simulink model "afe_uvw_ctrl"  (R2026b)
settings: Solver=VariableStepAuto
undefined symbols (not defined in the file or in its folder): param
(part 1 of 2)
settings Model: Creator=pwr-control  LastModifiedBy=d.bagnara

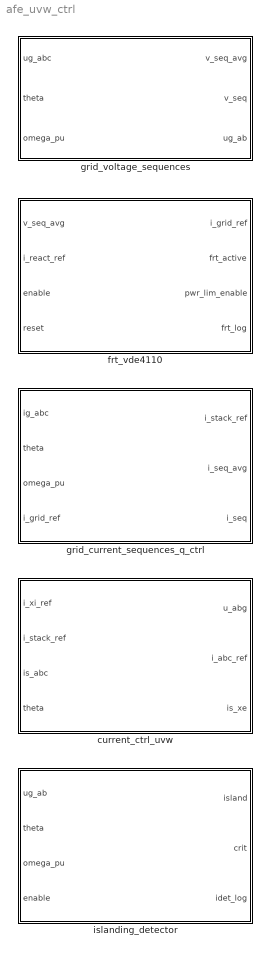
== system afe_uvw_ctrl ==
  current_ctrl_uvw : Subsystem  mask(Per-phase resonant current control (MATLAB Function)){p=param.afe.uvw}
      mask prompts: p "Parameter struct p (see afe_uvw_ctrl_param_example.m)"
      mask help: Current control of the stack (converter) current, one resonant PI per phase: the references of the sequence frames (xi from the DC-link control, [pos_eta; neg_xi; neg_eta] from grid_current_sequences_q_ctrl) become three phase current references; per phase d = kp*e + ki*s/(s^2 + 2*delta*w*s + w^2)*e (forward-backward Euler with p.ts: the new x1 in the update of x2, poles inside the unit circle for delta greater than 0; w = p.ictrl.omega_res, delta = p.ictrl.delta_res); the three outputs are divided by the length of the previous alpha/beta vector (limited to [p.ictrl.mag_lim, p.ictrl.mag_scale_max]) and transformed to alpha/beta, one step late as the model when p.ictrl.out_delay = 1; a PI on the zero-sequence current gives u_gamma. Inputs: i_xi_ref [pu], i_stack_ref [3x1] pu, is_abc [3x1] pu, theta [rad]. Outputs: u_abg [3x1] = [u_alpha; u_beta; u_gamma] pu for the modulator, i_abc_ref [3x1] pu, is_xe [2x1] = [xi; eta] stack current in the positive frame (log). MATLAB Function version of the subsystem current_ctrl of the model afe_uvw_three_phase. Source src/current_ctrl_uvw.m of library/masked_models/afe_uvw_ctrl (update_afe_uvw_ctrl.m loads it into the block). The block inherits its sample time: run it at p.ts (triggered or discrete subsystem clocked at p.ts, as the control of the model, or a fixed-step discrete model). Parameter p: one struct for the five blocks, see afe_uvw_ctrl_param_example.m. User guide: Help of the block (README.md of the folder).
      mask Help: web('https://github.com/pwr-control/library/blob/dev/library/masked_models/afe_uvw_ctrl/README.md', '-browser')
      mask Display:
      | disp(sprintf('per-phase resonant\ncurrent control'))
      | port_label('input', 1, 'i_xi_ref')
      | port_label('input', 2, 'i_stack_ref')
      | port_label('input', 3, 'is_abc')
      | port_label('input', 4, 'theta')
      | port_label('output', 1, 'u_abg')
      | port_label('output', 2, 'i_abc_ref')
      | port_label('output', 3, 'is_xe')
  frt_vde4110 : Subsystem  mask(Fault ride-through VDE-AR-N 4110 (MATLAB Function)){p=param.afe.uvw}
      mask prompts: p "Parameter struct p (see afe_uvw_ctrl_param_example.m)"
      mask help: Fault detection and reactive current references for the fault ride-through. A fault is detected when the positive sequence leaves [p.frt.v_pos_low, p.frt.v_pos_high] or the negative sequence exceeds p.frt.v_neg_max while the voltage changes faster than p.frt.v_pos_dot_max (double-integrator observers); state machine IDLE / ACTIVE / EXCEEDED (fault longer than p.frt.t_hold_max, left with reset). During the fault: pwr_lim_enable when the voltage is below p.frt.pwrlim_v_pos, and i_grid_ref = [pos_eta; neg_xi; neg_eta] = normal reactive references + p.frt.k_frt_ref times the change of the voltage sequences against their pre-fault averages (p.frt.t_avg_prefault, frozen during the fault), limited and low-pass filtered (p.frt.f_lpf_ref). Inputs: v_seq_avg [4x1] from grid_voltage_sequences, i_react_ref [2x1] = [pos; neg] reactive grid current references in normal operation [pu], enable (> 0.5 detector on), reset (> 0.5 leaves EXCEEDED). Outputs: i_grid_ref [3x1] pu -> grid_current_sequences_q_ctrl, frt_active (0/1), pwr_lim_enable (0/1, for the DC-link control), frt_log [10x1] = [state; exceeded; red_dyn; v_pos_dot; v_neg_dot; v_prefault (4); |v_neg|]. MATLAB Function version of the subsystem FRT-VDE4110 of the model afe_uvw_three_phase. Source src/frt_vde4110.m of library/masked_models/afe_uvw_ctrl (update_afe_uvw_ctrl.m loads it into the block). The block inherits its sample time: run it at p.ts (triggered or discrete subsystem clocked at p.ts, as the control of the model, or a fixed-step discrete model). Parameter p: one struct for the five blocks, see afe_uvw_ctrl_param_example.m. User guide: Help of the block (README.md of the folder).
      mask Help: web('https://github.com/pwr-control/library/blob/dev/library/masked_models/afe_uvw_ctrl/README.md', '-browser')
      mask Display:
      | disp(sprintf('fault ride-through\nVDE-AR-N 4110'))
      | port_label('input', 1, 'v_seq_avg')
      | port_label('input', 2, 'i_react_ref')
      | port_label('input', 3, 'enable')
      | port_label('input', 4, 'reset')
      | port_label('output', 1, 'i_grid_ref')
      | port_label('output', 2, 'frt_active')
      | port_label('output', 3, 'pwr_lim_enable')
      | port_label('output', 4, 'frt_log')
  grid_current_sequences_q_ctrl : Subsystem  mask(Grid current sequences and reactive current control (MATLAB Function)){p=param.afe.uvw}
      mask prompts: p "Parameter struct p (see afe_uvw_ctrl_param_example.m)"
      mask help: Sequence components of the grid current (same transformation and moving average as grid_voltage_sequences) and three PI controllers with clamped integrators that make the averaged positive-sequence eta and negative-sequence xi and eta grid currents follow i_grid_ref; the outputs are the stack current references for current_ctrl_uvw. Error = p.iseq.err_sign * (reference - measured): err_sign = -1 when the grid current is measured towards the converter (the model), +1 otherwise. Inputs: ig_abc [3x1] pu, theta [rad], omega_pu [pu], i_grid_ref [3x1] = [pos_eta; neg_xi; neg_eta] pu (frt_vde4110). Outputs: i_stack_ref [3x1] = [pos_eta; neg_xi; neg_eta] pu, i_seq_avg [4x1] = [pos_xi; pos_eta; neg_xi; neg_eta] averaged, i_seq [4x1] unfiltered. MATLAB Function version of the subsystem grid_current_sequences_and_reactive_pwr_ctrl of the model afe_uvw_three_phase. Source src/grid_current_sequences_q_ctrl.m of library/masked_models/afe_uvw_ctrl (update_afe_uvw_ctrl.m loads it into the block). The block inherits its sample time: run it at p.ts (triggered or discrete subsystem clocked at p.ts, as the control of the model, or a fixed-step discrete model). Parameter p: one struct for the five blocks, see afe_uvw_ctrl_param_example.m. User guide: Help of the block (README.md of the folder).
      mask Help: web('https://github.com/pwr-control/library/blob/dev/library/masked_models/afe_uvw_ctrl/README.md', '-browser')
      mask Display:
      | disp(sprintf('grid current sequences\nreactive current control'))
      | port_label('input', 1, 'ig_abc')
      | port_label('input', 2, 'theta')
      | port_label('input', 3, 'omega_pu')
      | port_label('input', 4, 'i_grid_ref')
      | port_label('output', 1, 'i_stack_ref')
      | port_label('output', 2, 'i_seq_avg')
      | port_label('output', 3, 'i_seq')
  grid_voltage_sequences : Subsystem  mask(Grid voltage sequences (MATLAB Function)){p=param.afe.uvw}
      mask prompts: p "Parameter struct p (see afe_uvw_ctrl_param_example.m)"
      mask help: Positive- and negative-sequence components of the grid voltage in the frames turned by +theta and -theta (xi/eta), averaged over a window of grid period / p.vseq.avg_order that follows the measured pulsation (half period with avg_order 2: the 100 Hz ripple of the other sequence is removed). Inputs: ug_abc [3x1] pu, theta [rad] angle of the PLL, omega_pu [pu] pulsation of the PLL. Outputs: v_seq_avg [4x1] = [pos_xi; pos_eta; neg_xi; neg_eta] averaged (zero before p.vseq.t_enable), v_seq [4x1] the same unfiltered, ug_ab [2x1] = [alpha; beta] (Clarke, amplitude invariant). MATLAB Function version of the subsystem grid_voltage_sequences of the model afe_uvw_three_phase (pwr-control/modelization-and-control). Source src/grid_voltage_sequences.m of library/masked_models/afe_uvw_ctrl (update_afe_uvw_ctrl.m loads it into the block). The block inherits its sample time: run it at p.ts (triggered or discrete subsystem clocked at p.ts, as the control of the model, or a fixed-step discrete model). Parameter p: one struct for the five blocks, see afe_uvw_ctrl_param_example.m. User guide: Help of the block (README.md of the folder).
      mask Help: web('https://github.com/pwr-control/library/blob/dev/library/masked_models/afe_uvw_ctrl/README.md', '-browser')
      mask Display:
      | disp(sprintf('grid voltage\nsequences'))
      | port_label('input', 1, 'ug_abc')
      | port_label('input', 2, 'theta')
      | port_label('input', 3, 'omega_pu')
      | port_label('output', 1, 'v_seq_avg')
      | port_label('output', 2, 'v_seq')
      | port_label('output', 3, 'ug_ab')
  islanding_detector : Subsystem  mask(Passive islanding detector (MATLAB Function)){p=param.afe.uvw}
      mask prompts: p "Parameter struct p (see afe_uvw_ctrl_param_example.m)"
      mask help: Passive islanding detection from the grid voltage and the PLL frequency: six criteria, each with its threshold and its on-delay (the condition must hold for the whole delay): under-voltage (p.island.u_min, t_trip_u_min), over-voltage (u_max, t_trip_u_max), under- and over-frequency (f_min, f_max, t_trip_f), rate of change of frequency (rocof_max [Hz/s], t_trip_rocof, from a double-integrator observer on the PLL pulsation) and voltage harmonics sqrt(u5^2 + u7^2)/u1 > h_max (t_trip_h). The frequency and harmonic criteria are blocked below p.island.u_valid (a grid fault is handled by frt_vde4110). Output latched until enable = 0 when p.island.latch = 1. Inputs: ug_ab [2x1] = [alpha; beta] pu (grid_voltage_sequences), theta [rad], omega_pu [pu], enable (0 also resets). Outputs: island (0/1), crit = bit mask of the criteria that tripped (1 U<, 2 U>, 4 f<, 8 f>, 16 ROCOF, 32 harmonics), idet_log [8x1] = [u1; u5; u7; harmonic ratio; f [pu]; ROCOF [Hz/s]; longest running criterion [s]; time since detection [s]]. New block: the model only measures the 7th harmonic. Source src/islanding_detector.m of library/masked_models/afe_uvw_ctrl (update_afe_uvw_ctrl.m loads it into the block). The block inherits its sample time: run it at p.ts (triggered or discrete subsystem clocked at p.ts, as the control of the model, or a fixed-step discrete model). Parameter p: one struct for the five blocks, see afe_uvw_ctrl_param_example.m. User guide: Help of the block (README.md of the folder).
      mask Help: web('https://github.com/pwr-control/library/blob/dev/library/masked_models/afe_uvw_ctrl/README.md', '-browser')
      mask Display:
      | disp(sprintf('islanding detector\n(passive)'))
      | port_label('input', 1, 'ug_ab')
      | port_label('input', 2, 'theta')
      | port_label('input', 3, 'omega_pu')
      | port_label('input', 4, 'enable')
      | port_label('output', 1, 'island')
      | port_label('output', 2, 'crit')
      | port_label('output', 3, 'idet_log')

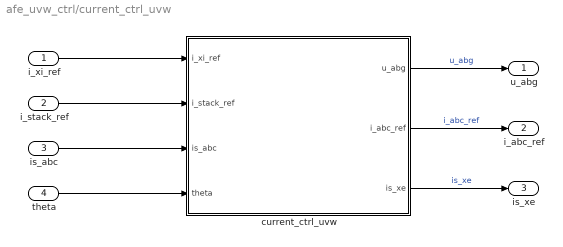
== system afe_uvw_ctrl/current_ctrl_uvw ==
  i_xi_ref : Inport
  i_stack_ref : Inport  Port=2
  is_abc : Inport  Port=3
  theta : Inport  Port=4
  current_ctrl_uvw : MATLAB Function  TreatAsAtomicUnit=on
  u_abg : Outport  VectorParamsAs1DForOutWhenUnconnected=off
  i_abc_ref : Outport  Port=2  VectorParamsAs1DForOutWhenUnconnected=off
  is_xe : Outport  Port=3  VectorParamsAs1DForOutWhenUnconnected=off
  wires:
  i_xi_ref/1 -> current_ctrl_uvw/1(i_xi_ref)
  i_stack_ref/1 -> current_ctrl_uvw/2(i_stack_ref)
  is_abc/1 -> current_ctrl_uvw/3(is_abc)
  theta/1 -> current_ctrl_uvw/4(theta)
  current_ctrl_uvw/1(u_abg) -> u_abg/1  "u_abg"
  current_ctrl_uvw/2(i_abc_ref) -> i_abc_ref/1  "i_abc_ref"
  current_ctrl_uvw/3(is_xe) -> is_xe/1  "is_xe"

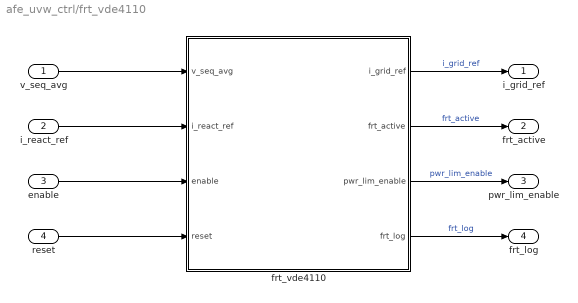
== system afe_uvw_ctrl/frt_vde4110 ==
  v_seq_avg : Inport
  i_react_ref : Inport  Port=2
  enable : Inport  Port=3
  reset : Inport  Port=4
  frt_vde4110 : MATLAB Function  TreatAsAtomicUnit=on
  i_grid_ref : Outport  VectorParamsAs1DForOutWhenUnconnected=off
  frt_active : Outport  Port=2  VectorParamsAs1DForOutWhenUnconnected=off
  pwr_lim_enable : Outport  Port=3  VectorParamsAs1DForOutWhenUnconnected=off
  frt_log : Outport  Port=4  VectorParamsAs1DForOutWhenUnconnected=off
  wires:
  v_seq_avg/1 -> frt_vde4110/1(v_seq_avg)
  i_react_ref/1 -> frt_vde4110/2(i_react_ref)
  enable/1 -> frt_vde4110/3(enable)
  reset/1 -> frt_vde4110/4(reset)
  frt_vde4110/1(i_grid_ref) -> i_grid_ref/1  "i_grid_ref"
  frt_vde4110/2(frt_active) -> frt_active/1  "frt_active"
  frt_vde4110/3(pwr_lim_enable) -> pwr_lim_enable/1  "pwr_lim_enable"
  frt_vde4110/4(frt_log) -> frt_log/1  "frt_log"

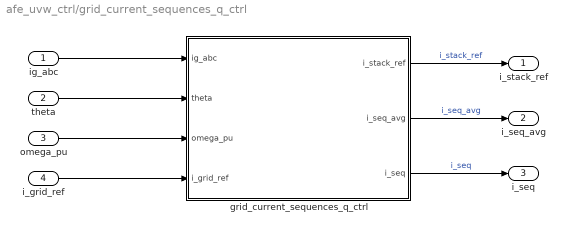
== system afe_uvw_ctrl/grid_current_sequences_q_ctrl ==
  ig_abc : Inport
  theta : Inport  Port=2
  omega_pu : Inport  Port=3
  i_grid_ref : Inport  Port=4
  grid_current_sequences_q_ctrl : MATLAB Function  TreatAsAtomicUnit=on
  i_stack_ref : Outport  VectorParamsAs1DForOutWhenUnconnected=off
  i_seq_avg : Outport  Port=2  VectorParamsAs1DForOutWhenUnconnected=off
  i_seq : Outport  Port=3  VectorParamsAs1DForOutWhenUnconnected=off
  wires:
  ig_abc/1 -> grid_current_sequences_q_ctrl/1(ig_abc)
  theta/1 -> grid_current_sequences_q_ctrl/2(theta)
  omega_pu/1 -> grid_current_sequences_q_ctrl/3(omega_pu)
  i_grid_ref/1 -> grid_current_sequences_q_ctrl/4(i_grid_ref)
  grid_current_sequences_q_ctrl/1(i_stack_ref) -> i_stack_ref/1  "i_stack_ref"
  grid_current_sequences_q_ctrl/2(i_seq_avg) -> i_seq_avg/1  "i_seq_avg"
  grid_current_sequences_q_ctrl/3(i_seq) -> i_seq/1  "i_seq"

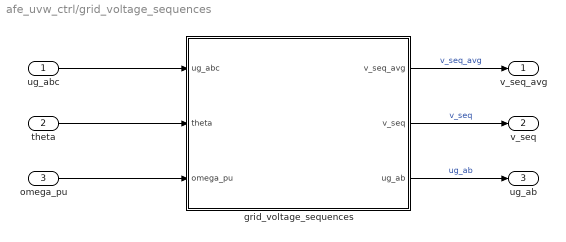
== system afe_uvw_ctrl/grid_voltage_sequences ==
  ug_abc : Inport
  theta : Inport  Port=2
  omega_pu : Inport  Port=3
  grid_voltage_sequences : MATLAB Function  TreatAsAtomicUnit=on
  v_seq_avg : Outport  VectorParamsAs1DForOutWhenUnconnected=off
  v_seq : Outport  Port=2  VectorParamsAs1DForOutWhenUnconnected=off
  ug_ab : Outport  Port=3  VectorParamsAs1DForOutWhenUnconnected=off
  wires:
  ug_abc/1 -> grid_voltage_sequences/1(ug_abc)
  theta/1 -> grid_voltage_sequences/2(theta)
  omega_pu/1 -> grid_voltage_sequences/3(omega_pu)
  grid_voltage_sequences/1(v_seq_avg) -> v_seq_avg/1  "v_seq_avg"
  grid_voltage_sequences/2(v_seq) -> v_seq/1  "v_seq"
  grid_voltage_sequences/3(ug_ab) -> ug_ab/1  "ug_ab"

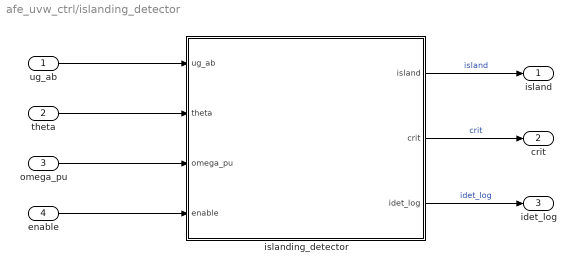
== system afe_uvw_ctrl/islanding_detector ==
  ug_ab : Inport
  theta : Inport  Port=2
  omega_pu : Inport  Port=3
  enable : Inport  Port=4
  islanding_detector : MATLAB Function  TreatAsAtomicUnit=on
  island : Outport  VectorParamsAs1DForOutWhenUnconnected=off
  crit : Outport  Port=2  VectorParamsAs1DForOutWhenUnconnected=off
  idet_log : Outport  Port=3  VectorParamsAs1DForOutWhenUnconnected=off
  wires:
  ug_ab/1 -> islanding_detector/1(ug_ab)
  theta/1 -> islanding_detector/2(theta)
  omega_pu/1 -> islanding_detector/3(omega_pu)
  enable/1 -> islanding_detector/4(enable)
  islanding_detector/1(island) -> island/1  "island"
  islanding_detector/2(crit) -> crit/1  "crit"
  islanding_detector/3(idet_log) -> idet_log/1  "idet_log"

== matlab function afe_uvw_ctrl/grid_voltage_sequences/grid_voltage_sequences ==
  data: ug_abc input size=[3 1]; theta input size=1; omega_pu input size=1; v_seq_avg output size=[4 1]; v_seq output size=[4 1]; ug_ab output size=[2 1]; p parameter
function [v_seq_avg, v_seq, ug_ab] = grid_voltage_sequences(ug_abc, theta, omega_pu, p)
%GRID_VOLTAGE_SEQUENCES  Positive and negative sequence of the grid voltage (xi, eta frames).
%
%   [v_seq_avg, v_seq, ug_ab] = grid_voltage_sequences(ug_abc, theta, omega_pu, p)
%
%   MATLAB Function version of the subsystem grid_voltage_sequences of the model afe_uvw_three_phase
%   (afe_uvw_ctrl.slx, pwr-control/modelization-and-control). Three steps:
%     1. Clarke transformation abc -> alpha, beta (amplitude invariant, factor 2/3);
%     2. rotation with the PLL angle into the positive-sequence frame and into the negative-sequence
%        frame (xi, eta);
%     3. moving average of the four components over a window that follows the grid frequency.
%
%   Inputs
%     ug_abc    [3x1] grid phase voltages [pu]
%     theta     grid angle of the PLL [rad]              (phase_grid_pll in the model)
%     omega_pu  grid pulsation of the PLL [pu of p.omega_nom] (omega_grid_pll_pu in the model)
%     p         parameter struct, see afe_uvw_ctrl_param_example.m: p.ts, p.omega_nom, p.vseq.*
%
%   Outputs
%     v_seq_avg [4x1] [pos_xi; pos_eta; neg_xi; neg_eta] after the moving average
%                     (v_grid_pos_xi_avg, v_grid_pos_eta_avg, v_grid_neg_xi_avg, v_grid_neg_eta_avg)
%     v_seq     [4x1] the same components before the average
%     ug_ab     [2x1] [alpha; beta] of the grid voltage [pu] (ug_alpha_pu, ug_beta_pu)
%
%   Frames (convention of the model)
%     positive: xi =  alpha*cos(theta) + beta*sin(theta),   eta = -alpha*sin(theta) + beta*cos(theta)
%     negative: xi =  alpha*cos(theta) - beta*sin(theta),   eta =  alpha*sin(theta) + beta*cos(theta)
%   With theta locked to the positive sequence, the positive sequence is a constant vector in the
%   positive frame and a vector rotating at 2*omega in the negative frame (and the other way round for
%   the negative sequence): the moving average over half a grid period (p.vseq.avg_order = 2) removes
%   the 2*omega term exactly, over a full period (avg_order = 1) it removes every harmonic as well.
%
%   Discrete time
%     The function runs once per control period p.ts (inside the triggered control subsystem, or with
%     the block sample time set to p.ts). Averaging window T = 2*pi/(p.omega_nom*p.vseq.avg_order*w),
%     with w = |omega_pu| limited to [p.vseq.omega_pu_min, p.vseq.omega_pu_max]. N = T/p.ts is not an
%     integer: the window holds floor(N) whole samples plus the next older one with the fractional
%     weight (see moving_average_frac at the end of this file). Before p.vseq.t_enable the averages are
%     zero (as the dmavg_flt blocks of the model); from then on they are the mean of the samples
%     received so far, until the window is full.
%
%   States (persistent)
%     buf       [4 x N_BUF] circular buffer of the last samples of v_seq
%     idx       position of the newest sample in buf
%     n_filled  number of valid samples in buf (saturates at N_BUF)
%     n_call    number of calls since the start (start-up delay t_enable = n_call*ts)
%
%   See also grid_current_sequences_q_ctrl, frt_vde4110, afe_uvw_ctrl_param_example.

    N_BUF = 4096;                    % buffer length [samples]; must be >= the longest window + 1
                                     % (window at omega_pu_min: 2*pi/(omega_nom*avg_order*omega_pu_min)/ts)

    persistent buf idx n_filled n_call
    if isempty(buf)
        buf = zeros(4, N_BUF);
        idx = 0;
        n_filled = 0;
        n_call = 0;
    end

    % ---- 1. Clarke transformation, amplitude invariant
    alpha = 2/3*(ug_abc(1) - 0.5*ug_abc(2) - 0.5*ug_abc(3));
    beta  = 1/sqrt(3)*(ug_abc(2) - ug_abc(3));
    ug_ab = [alpha; beta];

    % ---- 2. rotation into the positive and the negative sequence frame
    c = cos(theta);
    s = sin(theta);
    pos_xi  =  alpha*c + beta*s;
    pos_eta = -alpha*s + beta*c;
    neg_xi  =  alpha*c - beta*s;
    neg_eta =  alpha*s + beta*c;
    v_seq = [pos_xi; pos_eta; neg_xi; neg_eta];

    % ---- 3. moving average over T = 2*pi/(avg_order*omega) with the measured grid pulsation
    w = min(max(abs(omega_pu), p.vseq.omega_pu_min), p.vseq.omega_pu_max);
    T_avg = 2*pi/(p.omega_nom*p.vseq.avg_order*w);           % [s] averaging window
    n_win = min(T_avg/p.ts, N_BUF - 1);                       % [samples], not an integer

    n_call = n_call + 1;
    if (n_call - 1)*p.ts >= p.vseq.t_enable - 0.5*p.ts        % t = (n_call-1)*ts >= t_enable
        [v_seq_avg, buf, idx, n_filled] = moving_average_frac(v_seq, n_win, buf, idx, n_filled);
    else
        v_seq_avg = zeros(4, 1);                              % start-up: averages off (as the model)
    end
end


function [y, buf, idx, n_filled] = moving_average_frac(u, n_win, buf, idx, n_filled)
%MOVING_AVERAGE_FRAC  Moving average of the column vector u over a window of n_win samples (real).
%   The newest sample u is written into the circular buffer buf (one row per channel), idx is moved
%   to it. The window holds n_whole = floor(n_win) samples, the newest first, plus the next older one
%   with the weight frac = n_win - n_whole, so that the window length follows the grid period without
%   jumps. During the start-up (fewer samples than the window) the mean of the stored samples is used.
    n_buf = size(buf, 2);

    idx = idx + 1;
    if idx > n_buf
        idx = 1;
    end
    buf(:, idx) = u;
    n_filled = min(n_filled + 1, n_buf);

    n_whole = floor(n_win);
    frac = n_win - n_whole;
    if n_filled <= n_whole                 % not enough samples yet for the whole window
        n_whole = n_filled;
        frac = 0;
    end

    acc = zeros(size(u));
    j = idx;
    for k = 1:n_whole                      % the n_whole newest samples
        acc = acc + buf(:, j);
        j = j - 1;
        if j < 1
            j = n_buf;
        end
    end
    acc = acc + frac*buf(:, j);            % the next older sample, fractional weight
    y = acc/(n_whole + frac);
end

== matlab function afe_uvw_ctrl/frt_vde4110/frt_vde4110 ==
  data: v_seq_avg input size=[4 1]; i_react_ref input size=[2 1]; enable input size=1; reset input size=1; i_grid_ref output size=[3 1]; frt_active output size=1; pwr_lim_enable output size=1; frt_log output size=[10 1]; p parameter
function [i_grid_ref, frt_active, pwr_lim_enable, frt_log] = frt_vde4110(v_seq_avg, i_react_ref, enable, reset, p)
%FRT_VDE4110  Fault ride-through (VDE-AR-N 4110): fault detection and reactive current references.
%
%   [i_grid_ref, frt_active, pwr_lim_enable, frt_log] = frt_vde4110(v_seq_avg, i_react_ref, enable, reset, p)
%
%   MATLAB Function version of the subsystem FRT-VDE4110 of the model afe_uvw_three_phase
%   (afe_uvw_ctrl.slx, pwr-control/modelization-and-control). Two parts:
%
%   A. Fault detection (the LVRT_detector of the model, plus its two voltage-rate observers).
%      State machine IDLE -> ACTIVE -> EXCEEDED:
%      - IDLE -> ACTIVE when the positive-sequence voltage leaves the band [v_pos_low, v_pos_high]
%        or the negative sequence exceeds v_neg_max, AND one of the two voltages is changing faster
%        than v_dot_max [pu/s], AND the detector has been idle for more than t_rearm;
%      - ACTIVE -> IDLE when the positive sequence is back inside the band narrowed by v_hyst;
%      - ACTIVE -> EXCEEDED after t_hold_max in ACTIVE (fault too long); EXCEEDED -> IDLE on reset.
%      In ACTIVE the power limitation flag is set when v_pos < pwrlim_v_pos or v_neg > pwrlim_v_neg
%      and released with hysteresis; the reduced dynamic support flag (red_dyn) is set when
%      p.frt.reddyn_enabled and the voltage is below reddyn_v_pos or the negative sequence above
%      reddyn_v_neg (the model has this input at 0).
%      The voltage rates are the velocity states of two linear double-integrator observers
%      (x' = v + kx*(u - x), v' = kv*(u - x), forward Euler, held at zero before t_obs_release):
%      the same algorithm as linear_double_integrator_observer_ccaller of the library.
%
%   B. Reactive current references (FRT-PosNegReactiveCurrentReferences of the model).
%      The pre-fault voltages are moving averages over t_avg_prefault (0.5 s) that are FROZEN while
%      the fault is active and start only at t_avg_start, when the sequence averages are valid (the
%      model's averages start at zero and take the start-up transient in); dv = v_seq_avg - v_prefault. During the fault
%          i_pos_eta = i_react_ref(1) + k_frt_ref*dv_pos_xi
%          i_neg_eta = i_react_ref(2) - k_frt_ref*dv_neg_xi
%          i_neg_xi  =                 k_frt_ref*dv_neg_eta
%      (the negative-sequence current is the negative-sequence voltage change turned by 90 degrees:
%      reactive current against the unbalance); outside the fault the first two are the inputs and
%      the third is zero. Each reference is limited to +-lim (the reduced limits lim_*_red when
%      red_dyn is active) and smoothed by a first-order low pass at f_lpf_ref (y = g0*u + g1*y,
%      g0 = 2*pi*f*ts, g1 = 1 - g0, as the u_161Hz_flt blocks of the model).
%
%   Inputs
%     v_seq_avg    [4x1] averaged grid voltage sequences [pos_xi; pos_eta; neg_xi; neg_eta] [pu]
%                        (output v_seq_avg of grid_voltage_sequences)
%     i_react_ref  [2x1] reactive current references in normal operation [pos; neg] [pu]
%                        (i_react_pos_ref, i_react_neg_ref of the model)
%     enable       > 0.5: detector enabled (the model: a step at settle_time when the FRT test is on)
%     reset        > 0.5: leaves the EXCEEDED state (the model: 1 for the first 25 ms)
%     p            parameter struct, see afe_uvw_ctrl_param_example.m: p.ts, p.frt.*
%
%   Outputs
%     i_grid_ref      [3x1] grid current references [pos_eta; neg_xi; neg_eta] [pu]
%                           (the bus i_grid_seq_ref of the model) -> grid_current_sequences_q_ctrl
%     frt_active      1 while the fault is detected
%     pwr_lim_enable  1 when the active power has to be limited (read by the DC-link controller)
%     frt_log         [10x1] [frt_state (0 idle, 1 active, 2 exceeded); frt_exceeded; red_dyn_active;
%                     vxi_p_dot; vxi_n_dot; v_prefault(4); |v_neg|]
%
%   States (persistent)
%     obs_x, obs_v  [2x1] observer states (position, velocity) for the positive and the negative xi
%     buf, idx, n_filled, acc   moving averages of the pre-fault voltages (4 channels, running sum)
%     y_lpf         [3x1] low-pass states of the three references
%     state, pwr_lim, n_active, n_idle   state machine, power-limit flag, sample counters
%     n_call        number of calls (time since the start = n_call*ts)
%
%   See also grid_voltage_sequences, grid_current_sequences_q_ctrl, afe_uvw_ctrl_param_example.

    N_BUF = 8192;                    % buffer of the pre-fault averages [samples] >= t_avg_prefault/ts

    IDLE = 0;  ACTIVE = 1;  EXCEEDED = 2;

    persistent obs_x obs_v buf idx n_filled acc y_lpf state pwr_lim n_active n_idle n_call
    if isempty(state)
        obs_x = zeros(2, 1);
        obs_v = zeros(2, 1);
        buf = zeros(4, N_BUF);
        idx = 0;
        n_filled = 0;
        acc = zeros(4, 1);
        y_lpf = zeros(3, 1);
        state = IDLE;
        pwr_lim = 0;
        n_active = 0;
        n_idle = 0;
        n_call = 0;
    end
    ts = p.ts;
    n_call = n_call + 1;
    t_now = (n_call - 1)*ts;

    v_pos_xi = v_seq_avg(1);
    v_neg_xi = v_seq_avg(3);
    v_neg_eta = v_seq_avg(4);
    v_neg = sqrt(v_neg_xi^2 + v_neg_eta^2);

    % ---- A1. voltage rate observers on the positive and the negative xi component
    if t_now < p.frt.t_obs_release - 0.5*ts       % observers held at zero at the start
        obs_x = zeros(2, 1);
        obs_v = zeros(2, 1);
    end
    u_obs = [v_pos_xi; v_neg_xi];
    e_obs = u_obs - obs_x;
    obs_x = obs_x + ts*(obs_v + p.frt.obs_kx*e_obs);
    obs_v = obs_v + ts*p.frt.obs_kv*e_obs;
    vxi_p_dot = abs(obs_v(1));
    vxi_n_dot = abs(obs_v(2));

    % ---- A2. fault detection state machine
    n_rearm = round(p.frt.t_rearm/ts);
    n_hold_max = round(p.frt.t_hold_max/ts);
    frt_exceeded = 0;
    red_dyn_active = 0;
    if enable > 0.5
        if state == IDLE
            out_of_band = v_pos_xi > p.frt.v_pos_high || v_pos_xi < p.frt.v_pos_low || v_neg > p.frt.v_neg_max;
            fast_change = vxi_p_dot > p.frt.v_pos_dot_max || vxi_n_dot > p.frt.v_neg_dot_max;
            if out_of_band && fast_change && n_idle > n_rearm
                state = ACTIVE;
            end
            frt_active = 0;
            n_active = 0;
            pwr_lim = 0;
            n_idle = n_idle + 1;

        elseif state == ACTIVE
            n_idle = 0;
            if v_pos_xi >= p.frt.v_pos_low + p.frt.v_hyst && v_pos_xi < p.frt.v_pos_high - p.frt.v_hyst
                state = IDLE;                       % voltage back in the band: fault over
            elseif n_active >= n_hold_max
                state = EXCEEDED;                   % fault too long
            end
            % power limitation
            if v_pos_xi < p.frt.pwrlim_v_pos || v_neg > p.frt.pwrlim_v_neg
                pwr_lim = 1;
            elseif v_pos_xi > p.frt.pwrlim_v_pos + p.frt.pwrlim_hyst && v_neg < p.frt.pwrlim_v_neg_release
                pwr_lim = 0;
            end
            % reduced dynamic grid support
            if p.frt.reddyn_enabled > 0.5 && (v_pos_xi < p.frt.reddyn_v_pos || v_neg > p.frt.reddyn_v_neg)
                red_dyn_active = 1;
            end
            frt_active = 1;
            n_active = n_active + 1;

        else                                            % EXCEEDED
            if reset > 0.5
                state = IDLE;
            end
            frt_exceeded = 1;
            frt_active = 0;
        end
        pwr_lim_enable = pwr_lim;
    else
        state = IDLE;
        frt_active = 0;
        pwr_lim_enable = 0;
    end
    frt_state = state;

    % ---- B1. pre-fault voltages: moving averages over t_avg_prefault, frozen during the fault
    n_avg = min(round(p.frt.t_avg_prefault/ts), N_BUF);
    if frt_active == 0 && t_now >= p.frt.t_avg_start - 0.5*ts   % not during the fault, not at the start
        [buf, idx, n_filled, acc] = moving_sum_push(v_seq_avg, n_avg, buf, idx, n_filled, acc);
    end
    if n_filled > 0
        v_prefault = acc/n_filled;
    else
        v_prefault = v_seq_avg;                              % nothing stored yet: no fault contribution
    end
    dv = v_seq_avg - v_prefault;

    % ---- B2. reactive current references
    if frt_active == 1
        i_pos_eta = i_react_ref(1) + p.frt.k_frt_ref*dv(1);
        i_neg_eta = i_react_ref(2) - p.frt.k_frt_ref*dv(3);
        i_neg_xi  =                  p.frt.k_frt_ref*dv(4);
    else
        i_pos_eta = i_react_ref(1);
        i_neg_eta = i_react_ref(2);
        i_neg_xi  = 0;
    end
    if red_dyn_active == 1
        lim = [p.frt.lim_pos_eta_red; p.frt.lim_neg_xi_red; p.frt.lim_neg_eta_red];
    else
        lim = [p.frt.lim_pos_eta; p.frt.lim_neg_xi; p.frt.lim_neg_eta];
    end
    i_raw = [i_pos_eta; i_neg_xi; i_neg_eta];
    i_raw = min(max(i_raw, -lim), lim);

    g0 = 2*pi*p.frt.f_lpf_ref*ts;                        % first-order low pass, forward Euler
    y_lpf = g0*i_raw + (1 - g0)*y_lpf;
    i_grid_ref = y_lpf;

    frt_log = [frt_state; frt_exceeded; red_dyn_active; vxi_p_dot; vxi_n_dot; v_prefault; v_neg];
end


function [buf, idx, n_filled, acc] = moving_sum_push(u, n_win, buf, idx, n_filled, acc)
%MOVING_SUM_PUSH  Push the sample u into the circular buffer and keep acc = sum of the last n_win.
%   buf [n_ch x n_buf], idx = position of the newest sample, n_filled = samples in the window
%   (at most n_win). The average is acc/n_filled.
    n_buf = size(buf, 2);
    idx = idx + 1;
    if idx > n_buf
        idx = 1;
    end
    if n_filled >= n_win                   % window full: the oldest sample leaves
        j = idx - n_win;
        if j < 1
            j = j + n_buf;
        end
        acc = acc - buf(:, j);
    else
        n_filled = n_filled + 1;
    end
    buf(:, idx) = u;
    acc = acc + u;
end

== matlab function afe_uvw_ctrl/grid_current_sequences_q_ctrl/grid_current_sequences_q_ctrl ==
  data: ig_abc input size=[3 1]; theta input size=1; omega_pu input size=1; i_grid_ref input size=[3 1]; i_stack_ref output size=[3 1]; i_seq_avg output size=[4 1]; i_seq output size=[4 1]; p parameter
function [i_stack_ref, i_seq_avg, i_seq] = grid_current_sequences_q_ctrl(ig_abc, theta, omega_pu, i_grid_ref, p)
%GRID_CURRENT_SEQUENCES_Q_CTRL  Sequences of the grid current and control of its reactive components.
%
%   [i_stack_ref, i_seq_avg, i_seq] = grid_current_sequences_q_ctrl(ig_abc, theta, omega_pu, i_grid_ref, p)
%
%   MATLAB Function version of the subsystem grid_current_sequences_and_reactive_pwr_ctrl of the model
%   afe_uvw_three_phase (afe_uvw_ctrl.slx, pwr-control/modelization-and-control), without the
%   Simulink / C-Caller selector. Two parts:
%     1. sequences of the grid current, exactly as grid_voltage_sequences does for the voltage:
%        Clarke, rotation into the positive and the negative frame with the PLL angle, moving average
%        over a window that follows the grid frequency;
%     2. three PI controllers that make the averaged grid current follow its references
%        (positive-sequence eta, negative-sequence xi and eta) by moving the references of the
%        stack (converter) current, which the inner current controller then tracks.
%   The positive-sequence xi (active) current is not controlled here: its reference comes from the
%   DC-link voltage controller.
%
%   Inputs
%     ig_abc      [3x1] grid phase currents [pu]
%     theta       grid angle of the PLL [rad]
%     omega_pu    grid pulsation of the PLL [pu of p.omega_nom]
%     i_grid_ref  [3x1] grid current references [pos_eta; neg_xi; neg_eta] [pu] (from frt_vde4110)
%     p           parameter struct, see afe_uvw_ctrl_param_example.m: p.ts, p.omega_nom, p.iseq.*
%
%   Outputs
%     i_stack_ref [3x1] stack current references [pos_eta; neg_xi; neg_eta] [pu]
%                       (i_stack_pos_eta_ref, i_stack_neg_xi_ref, i_stack_neg_eta_ref of the model)
%     i_seq_avg   [4x1] [pos_xi; pos_eta; neg_xi; neg_eta] averaged grid current
%                       (i_grid_pos_xi_avg ... i_grid_neg_eta_avg of the model)
%     i_seq       [4x1] the same before the average
%
%   Sign of the error. The model measures the grid current towards the converter and the stack
%   current out of the converter, so a grid eta current above its reference asks for MORE stack eta
%   current: the PI works on e = p.iseq.err_sign*(reference - measured) with err_sign = -1 (the model
%   has a Sum ref - meas followed by a gain -1). Set err_sign = +1 if the grid current of your model
%   is measured in the direction of the stack current.
%
%   PI controller (pi_clamped at the end of this file): u = kp*e + ui, ui = ui + ki*ts*e (backward
%   Euler), output limited to +-lim and the integral state clamped to u_lim - kp*e, which is the
%   anti-windup of the Simulink PI (unit delay fed with saturation - P). Gains and limits:
%   p.iseq.kp_pos, ki_pos, lim_pos_eta for the positive sequence; kp_neg, ki_neg, lim_neg_xi,
%   lim_neg_eta for the negative one (the model uses the positive limit for the negative xi too:
%   lim_neg_xi = ieta_pos_ref_lim, lim_neg_eta = ieta_neg_ref_lim).
%
%   Discrete time: one call per control period p.ts. Averaging window T = 2*pi/(p.omega_nom*
%   p.iseq.avg_order*w), w = |omega_pu| limited to [p.iseq.omega_pu_min, p.iseq.omega_pu_max];
%   averages zero before p.iseq.t_enable (as the dmavg_flt blocks of the model).
%
%   States (persistent)
%     buf, idx, n_filled, n_call   moving average, see grid_voltage_sequences
%     ui                           [3x1] integral states of the three PIs [pos_eta; neg_xi; neg_eta]
%
%   See also grid_voltage_sequences, frt_vde4110, current_ctrl_uvw, afe_uvw_ctrl_param_example.

    N_BUF = 4096;                    % buffer length [samples]; must be >= the longest window + 1

    persistent buf idx n_filled n_call ui
    if isempty(buf)
        buf = zeros(4, N_BUF);
        idx = 0;
        n_filled = 0;
        n_call = 0;
        ui = zeros(3, 1);
    end

    % ---- 1. sequences of the grid current
    alpha = 2/3*(ig_abc(1) - 0.5*ig_abc(2) - 0.5*ig_abc(3));
    beta  = 1/sqrt(3)*(ig_abc(2) - ig_abc(3));
    c = cos(theta);
    s = sin(theta);
    i_seq = [ alpha*c + beta*s;        % positive sequence xi
             -alpha*s + beta*c;        % positive sequence eta
              alpha*c - beta*s;        % negative sequence xi
              alpha*s + beta*c];       % negative sequence eta

    w = min(max(abs(omega_pu), p.iseq.omega_pu_min), p.iseq.omega_pu_max);
    T_avg = 2*pi/(p.omega_nom*p.iseq.avg_order*w);           % [s] averaging window
    n_win = min(T_avg/p.ts, N_BUF - 1);                       % [samples], not an integer

    n_call = n_call + 1;
    if (n_call - 1)*p.ts >= p.iseq.t_enable - 0.5*p.ts
        [i_seq_avg, buf, idx, n_filled] = moving_average_frac(i_seq, n_win, buf, idx, n_filled);
    else
        i_seq_avg = zeros(4, 1);
    end

    % ---- 2. reactive current control: averaged grid current -> stack current references
    e_pos_eta = p.iseq.err_sign*(i_grid_ref(1) - i_seq_avg(2));
    e_neg_xi  = p.iseq.err_sign*(i_grid_ref(2) - i_seq_avg(3));
    e_neg_eta = p.iseq.err_sign*(i_grid_ref(3) - i_seq_avg(4));

    [u_pos_eta, ui(1)] = pi_clamped(e_pos_eta, ui(1), p.iseq.kp_pos, p.iseq.ki_pos*p.ts, p.iseq.lim_pos_eta);
    [u_neg_xi,  ui(2)] = pi_clamped(e_neg_xi,  ui(2), p.iseq.kp_neg, p.iseq.ki_neg*p.ts, p.iseq.lim_neg_xi);
    [u_neg_eta, ui(3)] = pi_clamped(e_neg_eta, ui(3), p.iseq.kp_neg, p.iseq.ki_neg*p.ts, p.iseq.lim_neg_eta);

    i_stack_ref = [u_pos_eta; u_neg_xi; u_neg_eta];
end


function [u, ui] = pi_clamped(e, ui, kp, ki_ts, lim)
%PI_CLAMPED  PI controller with the integrator clamped to the output limit (anti-windup).
%   ui is the integral state; ki_ts = ki*ts. Backward Euler: the integral includes the present error.
    up = kp*e;
    ui = ui + ki_ts*e;
    u = min(max(up + ui, -lim), lim);
    ui = u - up;                      % when limited, the integral keeps what the limit leaves to it
end


function [y, buf, idx, n_filled] = moving_average_frac(u, n_win, buf, idx, n_filled)
%MOVING_AVERAGE_FRAC  Moving average of the column vector u over a window of n_win samples (real).
%   The newest sample u is written into the circular buffer buf (one row per channel), idx is moved
%   to it. The window holds n_whole = floor(n_win) samples, the newest first, plus the next older one
%   with the weight frac = n_win - n_whole, so that the window length follows the grid period without
%   jumps. During the start-up (fewer samples than the window) the mean of the stored samples is used.
    n_buf = size(buf, 2);

    idx = idx + 1;
    if idx > n_buf
        idx = 1;
    end
    buf(:, idx) = u;
    n_filled = min(n_filled + 1, n_buf);

    n_whole = floor(n_win);
    frac = n_win - n_whole;
    if n_filled <= n_whole                 % not enough samples yet for the whole window
        n_whole = n_filled;
        frac = 0;
    end

    acc = zeros(size(u));
    j = idx;
    for k = 1:n_whole                      % the n_whole newest samples
        acc = acc + buf(:, j);
        j = j - 1;
        if j < 1
            j = n_buf;
        end
    end
    acc = acc + frac*buf(:, j);            % the next older sample, fractional weight
    y = acc/(n_whole + frac);
end

== matlab function afe_uvw_ctrl/current_ctrl_uvw/current_ctrl_uvw ==
  data: i_xi_ref input size=1; i_stack_ref input size=[3 1]; is_abc input size=[3 1]; theta input size=1; u_abg output size=[3 1]; i_abc_ref output size=[3 1]; is_xe output size=[2 1]; p parameter
function [u_abg, i_abc_ref, is_xe] = current_ctrl_uvw(i_xi_ref, i_stack_ref, is_abc, theta, p)
%CURRENT_CTRL_UVW  Per-phase resonant current control of the AFE stack current (uvw frame).
%
%   [u_abg, i_abc_ref, is_xe] = current_ctrl_uvw(i_xi_ref, i_stack_ref, is_abc, theta, p)
%
%   MATLAB Function version of the subsystem current_ctrl of the model afe_uvw_three_phase
%   (afe_uvw_ctrl.slx, pwr-control/modelization-and-control). Four steps:
%     1. the current references of the sequence frames become three phase references: the positive
%        sequence (xi_ref, pos_eta_ref) turned by +theta, the negative one (neg_xi, neg_eta) by
%        -theta, summed in alpha/beta and transformed to abc;
%     2. one resonant PI per phase on e = i_ref - i_meas:
%            d = kp*e + ki * s/(s^2 + 2*delta*w*s + w^2) * e
%        with w = p.ictrl.omega_res (the grid pulsation) and the damping delta = p.ictrl.delta_res
%        (0 gives the ideal resonator kp + ki*s/(s^2 + w^2)). The resonator is in state-space form
%        x = [x1; x2], x1' = x2, x2' = -w^2*x1 - 2*delta*w*x2 + ki*e, output x2, and is discretized
%        with the step ts as forward Euler on x1 and backward Euler on x2 (the NEW x1 is used in the
%        update of x2):
%            x1+ = x1 + ts*x2,   x2+ = x2 + ts*(-w^2*x1+ - 2*delta*w*x2 + ki*e).
%        The discrete poles then have |z|^2 = 1 - 2*delta*w*ts: on the unit circle for delta = 0 and
%        inside it for delta > 0, with the resonance at w. The plain forward Euler of the model
%        (Aresd = I + A*ts, Bresd = B*ts, used by this block up to library rev. 02) has instead
%        |z|^2 = 1 - 2*delta*w*ts + (w*ts)^2, i.e. poles OUTSIDE the unit circle when delta < w*ts/2
%        (0.0196 at 125 us): with the model's delta = 0.015 that resonator alone is a growing
%        oscillator and its gain at w is 10.8 instead of ki/(2*delta*w) = 3.7. The loop with the plant
%        was still stable (the plant pulls the poles inside), but the damping now means what it says:
%        delta = 0.005 gives about the same gain at w (11.1 against 10.8) as the model's resonator with
%        0.015, and is the default of afe_uvw_ctrl_param_example.m;
%     3. vector limiter: the three outputs are divided by scale = |u_alpha_beta| of the previous
%        step, limited to [p.ictrl.mag_lim, p.ictrl.mag_scale_max] (the model's "antiwind_up"), so
%        that the voltage vector stays inside the unit circle; then abc -> alpha, beta (the zero
%        sequence of the three outputs is dropped). The model delivers alpha/beta through one Unit
%        Delay (p.ictrl.out_delay = 1 keeps that one-step delay, 0 removes it);
%     4. zero-sequence current control: PI with clamped integrator on p.ictrl.iz_ref - mean(is_abc),
%        output limited to +-p.ictrl.u_z_lim, gives u_gamma.
%
%   Inputs
%     i_xi_ref     positive-sequence xi (active) stack current reference [pu] (from the DC-link control)
%     i_stack_ref  [3x1] [pos_eta; neg_xi; neg_eta] stack current references [pu]
%                        (output of grid_current_sequences_q_ctrl)
%     is_abc       [3x1] stack (converter) phase currents [pu]
%     theta        grid angle of the PLL [rad]
%     p            parameter struct, see afe_uvw_ctrl_param_example.m: p.ts, p.ictrl.*
%
%   Outputs
%     u_abg        [3x1] [u_alpha; u_beta; u_gamma] voltage references for the modulator [pu]
%                        (ualpha_afe, ubeta_afe, ugamma_afe of the model)
%     i_abc_ref    [3x1] phase current references [pu] (isa_ref, isb_ref, isc_ref)
%     is_xe        [2x1] stack current in the positive frame [xi; eta] (id_xi_pu, id_eta_pu), for logging
%
%   States (persistent)
%     x_res   [2x3] resonator states of the three phases (columns a, b, c)
%     u_ab_d  [2x1] alpha/beta output of the previous step (vector limiter and output delay)
%     ui_z    integral state of the zero-sequence PI
%
%   See also grid_current_sequences_q_ctrl, afe_uvw_ctrl_param_example.

    persistent x_res u_ab_d ui_z
    if isempty(x_res)
        x_res = zeros(2, 3);
        u_ab_d = zeros(2, 1);
        ui_z = 0;
    end
    ts = p.ts;
    c = cos(theta);
    s = sin(theta);

    % ---- 1. references: sequence frames -> alpha/beta -> abc
    pos_xi = i_xi_ref;        pos_eta = i_stack_ref(1);
    neg_xi = i_stack_ref(2);  neg_eta = i_stack_ref(3);
    alpha_ref = (pos_xi*c - pos_eta*s) + (neg_xi*c + neg_eta*s);      % positive turned by +theta,
    beta_ref  = (pos_xi*s + pos_eta*c) + (-neg_xi*s + neg_eta*c);     % negative turned by -theta
    i_abc_ref = [alpha_ref;
                 -0.5*alpha_ref + sqrt(3)/2*beta_ref;
                 -0.5*alpha_ref - sqrt(3)/2*beta_ref];

    % ---- 2. resonant PI per phase (forward Euler on x1, backward Euler on x2)
    w = p.ictrl.omega_res;
    kp = p.ictrl.kp;
    ki = p.ictrl.ki;
    delta = p.ictrl.delta_res;
    e = i_abc_ref - is_abc;                                 % [3x1]
    d_abc = kp*e + x_res(2, :)';                            % output: P + resonator state x2
    x1 = x_res(1, :) + ts*x_res(2, :);                      % new x1 ...
    x2 = x_res(2, :) + ts*(-w^2*x1 - 2*delta*w*x_res(2, :) + ki*e');   % ... used in the update of x2
    x_res(1, :) = x1;
    x_res(2, :) = x2;

    % ---- 3. vector limiter on the previous output, abc -> alpha/beta, output delay
    scale = min(max(sqrt(u_ab_d(1)^2 + u_ab_d(2)^2), p.ictrl.mag_lim), p.ictrl.mag_scale_max);
    d_abc = d_abc/scale;
    u_ab = [2/3*(d_abc(1) - 0.5*d_abc(2) - 0.5*d_abc(3));
            1/sqrt(3)*(d_abc(2) - d_abc(3))];
    if p.ictrl.out_delay > 0.5
        u_ab_out = u_ab_d;                                  % as the model: one step late
    else
        u_ab_out = u_ab;
    end
    u_ab_d = u_ab;

    % ---- 4. zero-sequence current control
    iz = (is_abc(1) + is_abc(2) + is_abc(3))/3;
    e_z = p.ictrl.iz_ref - iz;
    up_z = p.ictrl.kp_z*e_z;
    ui_z = ui_z + p.ictrl.ki_z*ts*e_z;
    u_gamma = min(max(up_z + ui_z, -p.ictrl.u_z_lim), p.ictrl.u_z_lim);
    ui_z = u_gamma - up_z;                                  % integrator clamped to the limit

    u_abg = [u_ab_out; u_gamma];

    % ---- stack current in the positive frame, for logging
    is_alpha = 2/3*(is_abc(1) - 0.5*is_abc(2) - 0.5*is_abc(3));
    is_beta  = 1/sqrt(3)*(is_abc(2) - is_abc(3));
    is_xe = [ is_alpha*c + is_beta*s;
             -is_alpha*s + is_beta*c];
end
